simulink model "x3DOF_bener"  (R2024b)
settings: Solver=VariableStepAuto  StartTime=0.0  StopTime=250  FixedStep=au  RelTol=1e-10
undefined symbols (not defined in the file): controller, dr2, dr3, du2, du3, dv2, dv3, gamma, Gpi, guidance, IzMinNrd, m, magnitude, Nr, x_8, x_custom, x_elips, x_L, x_ling, x_s, x_sinus, Xu, Xud, y_8, y_custom, y_elips, y_L, y_ling, y_s, y_sinus, Yv, Yvd
libraries: fuzblock x8, simulink x6, mssSimulink x1
(part 1 of 2)
settings Model: PacingRate=1000  Creator=Baha'uddin  LastModifiedBy=User
settings DebuggingCC: UnderSpecifiedDimensionMsg=error

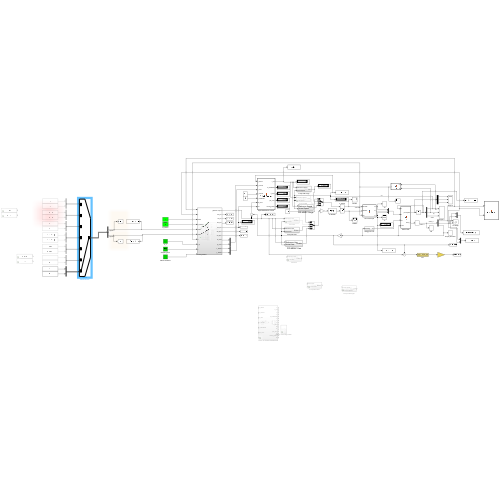
[thumbnail: Simulink's stored preview of the top-level diagram]
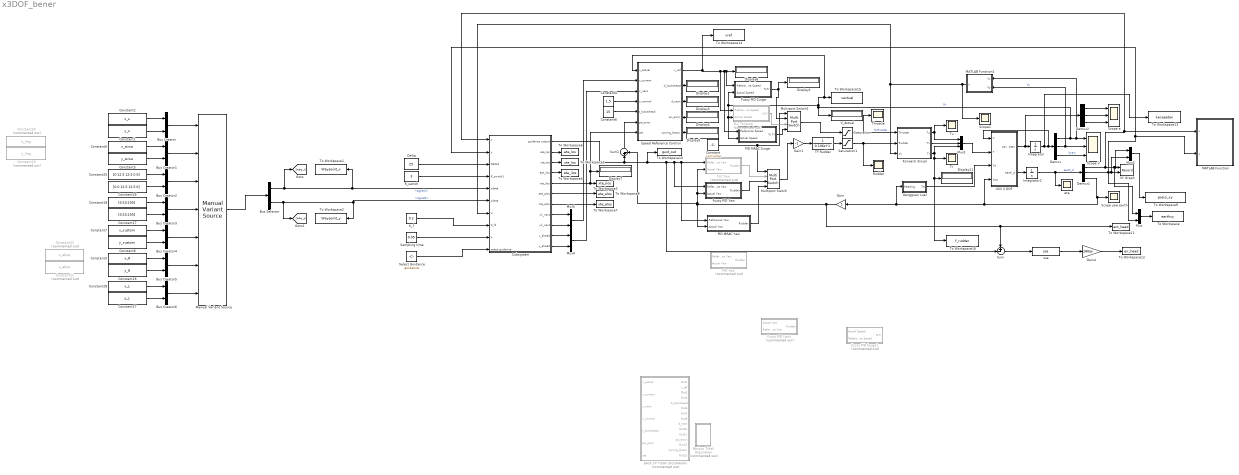
== system x3DOF_bener ==
  BACK UP TIDAK DIGUNAKAN : Subsystem  Commented=on
  Backup Tidak Digunakan : Subsystem  Commented=on
  Bus Creator{,1..6} (7 alike) : BusCreator  Inputs=2
  Bus Selector : BusSelector  OutputSignals=signal1,signal2
  Constant : Constant  Value=controller
  Constant1 : Constant  Value=y_s
  Constant16 : Constant  Value=y_8
  Constant17 : Constant  Value=[0:10:150]
  Constant18 : Constant  Value=[0:10:150]
  Constant2 : Constant  Value=x_s
  Constant21 : Constant  Commented=on  Value=y_elips
  Constant22 : Constant  Commented=on  Value=x_elips
  Constant23 : Constant  Commented=on  Value=y_ling
  Constant24 : Constant  Commented=on  Value=x_ling
  Constant25 : Constant  Value=[0 12.5 12.5 0 0]  VectorParams1D=off
  Constant26 : Constant  Value=[0 0 12.5 12.5 0]
  Constant27 : Constant  Value=y_L
  Constant28 : Constant  Value=x_L
  Constant3 : Constant  Value=x_8
  Constant4 : Constant  Value=1.5
  Constant5 : Constant  Value=y_sinus
  Constant6 : Constant  Value=15
  Constant7 : Constant  Value=x_custom
  Constant8 : Constant  Value=y_custom
  Constant9 : Constant  Value=x_sinus
  Delta : Constant  Value=25
  Demux : Demux  Outputs=3
  Demux1 : Demux  Outputs=3
  Demux2 : Demux  Outputs=3
  Display{1..7,11} (8 alike) : Display
  FLC Throttle : Subsystem  Commented=on
  FLC Yaw : Subsystem  Commented=on
  Fuzzy PID Surge : Subsystem
  Fuzzy PID Surge1 : Subsystem  Commented=on
  Fuzzy PID Yaw : Subsystem
  Fuzzy PID Yaw1 : Subsystem  Commented=on
  Gain : Gain
  Gain1 : Gain  Gain=-1
  Gain4 : Gain  Gain=180/pi
  Gangguan Luar : Subsystem
  Integrator : Integrator  InitialCondition=[0 0 0]
  Integrator2 : Integrator  InitialCondition=[0 0 deg2rad(0)]
  K_f : Constant  Value=0.2
  "Konversi Sinyal " : MATLAB Function  TreatAsAtomicUnit=on
  MATLAB Function : MATLAB Function  TreatAsAtomicUnit=on  SystemSampleTime=0.1
  MATLAB Function1 : MATLAB Function  TreatAsAtomicUnit=on
  Manual Variant Source : simulink/Signal Routing/Manual Variant Source  NumChoices=7  LabelModeActiveChoice=V_7
  Multiport Switch : MultiPortSwitch  SaturateOnIntegerOverflow=off  InputSameDT=off
  Multiport Switch1 : MultiPortSwitch  SaturateOnIntegerOverflow=off  InputSameDT=off
  Mux{,3..5} (4 alike) : Mux  Inputs=2
  Mux1 : Mux  Inputs=3
  PID MRAC Surge : Subsystem
  PID MRAC Yaw : Subsystem
  PID Yaw : Subsystem  Commented=on
  R_switch : Constant  Value=3
  Rudder : Scope
  Sampling time : Constant  Value=0.05
  Saturation : Saturate  UpperLimit=100  LowerLimit=0  ZeroCross=off
  Saturation1 : Saturate  UpperLimit=deg2rad(30)  LowerLimit=deg2rad(-30)
  Scope V : Scope  NumInputPorts=3
  Scope a : Scope  NumInputPorts=3
  Scope yaw earth : Scope
  Scope1 : Scope
  Select Guidance : Constant  Value=guidance
  Speed Reference Control : MATLAB Function  TreatAsAtomicUnit=on
  Subsystem : Subsystem
  Sum : Sum  Inputs=+-|
  Sum1 : Sum  Inputs=|+-
  TF Rudder : TransferFcn  Denominator=[0.106 1]
  Throttle : Scope
  To Workspace : ToWorkspace  VariableName=earthxy  SampleTime=-1
  To Workspace1 : ToWorkspace  VariableName=Waypoint_x  SampleTime=-1
  To Workspace10 : ToWorkspace  VariableName=guid_out  SaveFormat=Timeseries  SampleTime=0.05
      settings: Save2DSignal=2-D array (concatenate along first dimension)
  To Workspace11 : ToWorkspace  VariableName=act_head  SaveFormat=Timeseries  SampleTime=0.05
      settings: Save2DSignal=2-D array (concatenate along first dimension)
  To Workspace12 : ToWorkspace  VariableName=err_head  SaveFormat=Timeseries  SampleTime=0.05
      settings: Save2DSignal=2-D array (concatenate along first dimension)
  To Workspace13 : ToWorkspace  VariableName=kecepatan  SampleTime=1
  To Workspace14 : ToWorkspace  VariableName=vref  SampleTime=0.01
  To Workspace15 : ToWorkspace  VariableName=vactual  SampleTime=0.01
  To Workspace16 : ToWorkspace  VariableName=f_rudder  SampleTime=1
  To Workspace2 : ToWorkspace  VariableName=Waypoint_y  SampleTime=-1
  To Workspace3 : ToWorkspace  VariableName=xte_ilos  SaveFormat=Timeseries  SampleTime=0.05
  To Workspace4 : ToWorkspace  VariableName=ate_ilos  SaveFormat=Timeseries  SampleTime=0.05
  To Workspace5 : ToWorkspace  VariableName=xte_los  SaveFormat=Timeseries  SampleTime=0.05
      settings: Save2DSignal=2-D array (concatenate along first dimension)
  To Workspace6 : ToWorkspace  VariableName=ate_los  SaveFormat=Timeseries  SampleTime=0.05
      settings: Save2DSignal=2-D array (concatenate along first dimension)
  To Workspace7 : ToWorkspace  VariableName=xte_alos  SaveFormat=Timeseries  SampleTime=0.05
      settings: Save2DSignal=2-D array (concatenate along first dimension)
  To Workspace8 : ToWorkspace  VariableName=ate_alos  SaveFormat=Timeseries  SampleTime=0.05
      settings: Save2DSignal=2-D array (concatenate along first dimension)
  To Workspace9 : ToWorkspace  VariableName=posisi_xy  SampleTime=-1
      settings: Save2DSignal=2-D array (concatenate along first dimension)
  Tr : Scope
  Tu : Scope
  USV 3 DOF : MATLAB Function  TreatAsAtomicUnit=on
  V_Actual : Display
  XY Graph : Record  FileSettingsInternal="{\"entries\":[{\"content\":{\"excelSettings\":{\"content\":{},\"type\":\"Streamout.ExcelSettings\"}},\"type\":\"Streamout.FileSettingStorage\",\"uuid\":\"\"}],\"packageUris\":[\"http:\\/\\/schema.mathworks.com\\/mf0\\/streamout_blocks\\/R2020a\"],\"version\":\"1.0\"}"  Layout=[1 1]  SignalsInternal="{\"entries\":[{\"content\":{\"signals\":[{\"content\":{\"blockPath\":[],\"dimensions\":[1],\"domain\":\"\",\"lineColor\":\"#a2142f\",\"lineWidth\":2,\"port\":1,\"sid\":[\"\"],\"signalID\":1,\"signalName\":\"Demux1:1\"},\"type\":\"RecordBlkView.Signal\",\"uuid\":\"\"},{\"content\":{\"blockPath\":[],\"dimensions\":[1],\"domain\":\"\",\"lineColor\":\"#139fff\",\"lineWidth\":2,\"port\":2,\"sid\":[\"\"],\"signalID\":2,\"signalName\":\"Demux1:2\"},\"type\":\"RecordBlkView.Signal\",\"uuid\":\"\"}]},\"type\":\"RecordBlkView.InputSignals\",\"uuid\":\"\"}],\"packageUris\":[\"http:\\/\\/schema.mathworks.com\\/mf0\\/streamout_blocks\\/R2020a\"],\"version\":\"1.0\"}"  VisualizationBindings="{\"xyplotplugin\":{\"info\":[{\"series\":[],\"subplotID\":1}]}}"  CompatibilityTag=XY  st=-1
  eta : Scope
  "ssa " : mssSimulink/Utilities/Math Operations/ssa  SystemSampleTime=-1  VariantActivationTime=update diagram  AllowFlexibleInterface=on  Latency=0  AutoFrameSizeCalculation=off
  wires:
  Demux/3 -> Scope V/3  "Vyaw"
  Gangguan Luar/1(Te) -> USV 3 DOF/3(Te)
  USV 3 DOF/2(earth_d) -> Integrator2/1
  "Konversi Sinyal "/2(Tv) -> Mux1/2
  Mux1/1 -> USV 3 DOF/2(T)
  "Konversi Sinyal "/1(Tu) -> Mux1/1, Tu/1
  Integrator/1 -> To Workspace13/1, USV 3 DOF/1(V), Demux/1
  Demux/2 -> MATLAB Function1/2(Vy), Scope V/2  "Vy"
  Integrator2/1 -> Demux1/1, eta/1  "earth_d"
  "Konversi Sinyal "/3(Tr) -> To Workspace16/1, Display11/1, Tr/1, Mux1/3
  Saturation1/1 -> "Konversi Sinyal "/2(Rudder), Rudder/1
  Saturation/1 -> "Konversi Sinyal "/1(Throttle), Throttle/1  "%Throttle"
  USV 3 DOF/1(percepatan) -> Demux2/1, Integrator/1
  Demux2/1 -> Scope a/1
  Demux2/2 -> Scope a/2
  Demux2/3 -> Scope a/3
  Mux/1 -> To Workspace/1
  Gain/1 -> Sum/1, To Workspace11/1, PID MRAC Yaw/2(Actual Yaw), Sum1/2, FLC Yaw/2(Actual Yaw), Fuzzy PID Yaw/2(Actual Yaw)
  Subsystem/6(ate_alos) -> To Workspace8/1
  Subsystem/3(xte_los) -> To Workspace5/1
  Subsystem/7(xte_alos) -> To Workspace7/1
  Subsystem/4(ate_ilos) -> To Workspace4/1
  Subsystem/5(xte_ilos) -> Speed Reference Control/7(cte), Display7/1, To Workspace3/1
  Subsystem/2(ate_los) -> To Workspace6/1
  R_switch/1 -> Subsystem/4(R_switch1)
  K_f/1 -> Subsystem/8(K_f1)
  Delta/1 -> Subsystem/3(Delta1)
  Select Guidance/1 -> Subsystem/10(select guidance)
  Sampling time/1 -> Subsystem/9(h)
  Bus Selector/1 -> [way_x], To Workspace1/1, Subsystem/5(xdata)  "<signal1>"
  Bus Selector/2 -> [way_y], Subsystem/6(ydata), To Workspace2/1  "<signal2>"
  MATLAB Function1/1(y) -> "Konversi Sinyal "/3(Vx), Subsystem/7(U), Scope1/1
  Mux3/1 -> To Workspace9/1
  "ssa "/1 -> Gain4/1
  Gain4/1 -> To Workspace12/1
  Sum/1 -> "ssa "/1
  TF Rudder/1 -> Saturation1/1
  Demux/1 -> Speed Reference Control/1(v_actual), To Workspace15/1, PID MRAC Surge/2(Actual Speed), FLC Throttle/2(Actual Speed), Fuzzy PID Surge/2(Actual Speed), V_Actual/1, MATLAB Function1/1(Vx), Scope V/1  "Vx"
  Subsystem/10(x_ahead) -> Mux4/1
  Subsystem/11(y_ahead) -> Mux4/2
  Subsystem/8(xk_next) -> Mux5/1
  Subsystem/9(yk_next) -> Mux5/2
  Demux1/2 -> Subsystem/2(y), MATLAB Function/2(y), Mux/2, Mux3/2, XY Graph/2
  Subsystem/1(guidance output) -> To Workspace10/1, Sum/2, PID MRAC Yaw/1(Reference Yaw), FLC Yaw/1(Reference Yaw), Fuzzy PID Yaw/1(Reference Yaw), Sum1/1
  Demux1/3 -> USV 3 DOF/4(Yaw), Gain/1, Gangguan Luar/1(Heading), Scope yaw earth/1
  Demux1/1 -> Subsystem/1(x), MATLAB Function/1(x), Mux/1, Mux3/1, XY Graph/1
  Sum1/1 -> Speed Reference Control/6("psi_error ")
  Speed Reference Control/1(v_ref) -> FLC Throttle/1(Reference Speed), PID MRAC Surge/1(Reference Speed), Display6/1, Fuzzy PID Surge/1(Reference Speed), To Workspace14/1
  Speed Reference Control/2(d_lookahead) -> Display1/1
  Speed Reference Control/5(turning_factor) -> Display5/1
  Speed Reference Control/4(psi_error) -> Display4/1
  Speed Reference Control/3(d_next) -> Display3/1
  Gain1/1 -> TF Rudder/1
  Mux5/1 -> Speed Reference Control/2(x_current)
  Constant6/1 -> Speed Reference Control/5(t_lookahead)
  Constant4/1 -> Speed Reference Control/4(v_normal)
  Mux4/1 -> Speed Reference Control/3(x_next)
  Constant3/1 -> Bus Creator5/1
  Constant16/1 -> Bus Creator5/2
  Bus Creator1/1 -> Manual Variant Source/2
  Bus Creator2/1 -> Manual Variant Source/3
  Constant25/1 -> Bus Creator2/1
  Constant26/1 -> Bus Creator2/2
  Constant18/1 -> Bus Creator3/1
  Constant17/1 -> Bus Creator3/2
  Bus Creator3/1 -> Manual Variant Source/4
  Constant7/1 -> Bus Creator4/1
  Constant8/1 -> Bus Creator4/2
  Bus Creator4/1 -> Manual Variant Source/5
  Bus Creator5/1 -> Manual Variant Source/6
  Manual Variant Source/1 -> Bus Selector/1
  Bus Creator/1 -> Manual Variant Source/1
  Constant28/1 -> Bus Creator6/1
  Constant27/1 -> Bus Creator6/2
  Bus Creator6/1 -> Manual Variant Source/7
  FLC Yaw/1(Rudder) -> Multiport Switch/2
  Fuzzy PID Yaw/1(Rudder) -> Multiport Switch/3
  Constant/1 -> Multiport Switch1/1, Multiport Switch/1
  Multiport Switch/1 -> Gain1/1
  Fuzzy PID Surge/1(%Tr) -> Multiport Switch1/2, Display2/1
  FLC Throttle/1(%Tr) -> Multiport Switch1/3
  Constant2/1 -> Bus Creator/1
  Constant1/1 -> Bus Creator/2
  Constant9/1 -> Bus Creator1/1
  Constant5/1 -> Bus Creator1/2
  PID MRAC Yaw/1(Rudder) -> Multiport Switch/4
  Multiport Switch1/1 -> Saturation/1
  PID MRAC Surge/1(% Tr) -> Multiport Switch1/4

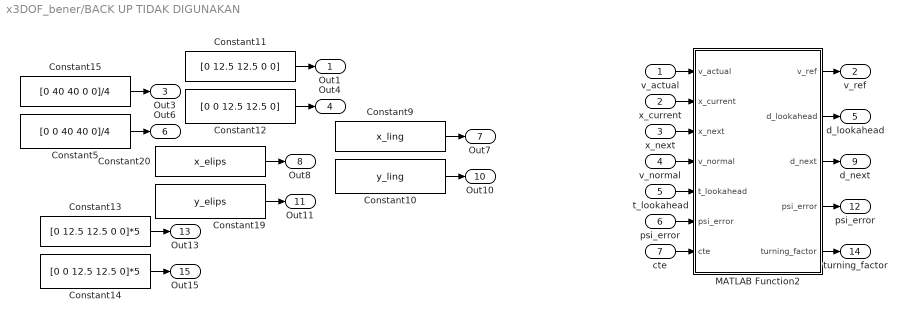
== system x3DOF_bener/BACK UP TIDAK DIGUNAKAN ==
  v_actual : Inport
  x_current : Inport  Port=2
  x_next : Inport  Port=3
  v_normal : Inport  Port=4
  t_lookahead : Inport  Port=5
  "psi_error " : Inport  Port=6
  cte : Inport  Port=7
  Constant10 : Constant  Value=y_ling
  Constant11 : Constant  Value=[0 12.5 12.5 0 0]  VectorParams1D=off
  Constant12 : Constant  Value=[0 0 12.5 12.5 0]
  Constant13 : Constant  Value=[0 12.5 12.5 0 0]*5  VectorParams1D=off
  Constant14 : Constant  Value=[0 0 12.5 12.5 0]*5
  Constant15 : Constant  Value=[0 40 40 0 0]/4  VectorParams1D=off
  Constant19 : Constant  Value=y_elips
  Constant20 : Constant  Value=x_elips
  Constant5 : Constant  Value=[0 0 40 40 0]/4
  Constant9 : Constant  Value=x_ling
  MATLAB Function2 : MATLAB Function  TreatAsAtomicUnit=on
  Out1 : Outport
  v_ref : Outport  Port=2
  Out3 : Outport  Port=3
  Out4 : Outport  Port=4
  d_lookahead : Outport  Port=5
  Out6 : Outport  Port=6
  Out7 : Outport  Port=7
  Out8 : Outport  Port=8
  d_next : Outport  Port=9
  Out10 : Outport  Port=10
  Out11 : Outport  Port=11
  psi_error : Outport  Port=12
  Out13 : Outport  Port=13
  turning_factor : Outport  Port=14
  Out15 : Outport  Port=15
  wires:
  Constant14/1 -> Out15/1
  Constant11/1 -> Out1/1
  Constant9/1 -> Out7/1
  Constant15/1 -> Out3/1
  Constant19/1 -> Out11/1
  Constant5/1 -> Out6/1
  Constant12/1 -> Out4/1
  Constant13/1 -> Out13/1
  Constant20/1 -> Out8/1
  t_lookahead/1 -> MATLAB Function2/5(t_lookahead)
  MATLAB Function2/4(psi_error) -> psi_error/1
  x_current/1 -> MATLAB Function2/2(x_current)
  v_normal/1 -> MATLAB Function2/4(v_normal)
  x_next/1 -> MATLAB Function2/3(x_next)
  "psi_error "/1 -> MATLAB Function2/6("psi_error ")
  cte/1 -> MATLAB Function2/7(cte)
  MATLAB Function2/1(v_ref) -> v_ref/1
  MATLAB Function2/3(d_next) -> d_next/1
  MATLAB Function2/2(d_lookahead) -> d_lookahead/1
  MATLAB Function2/5(turning_factor) -> turning_factor/1
  Constant10/1 -> Out10/1
  v_actual/1 -> MATLAB Function2/1(v_actual)

== system x3DOF_bener/Backup Tidak Digunakan ==
  3 DOF : Subsystem  Commented=on
  From Workspace2 : FromWorkspace  Commented=on  VariableName=THR_ts  SampleTime=0.001
  From Workspace3 : FromWorkspace  Commented=on  VariableName=STER_ts  SampleTime=0.001
  Gangguan Luar1 : Subsystem  Commented=on
  Konversi Sinyal 1 : MATLAB Function  Commented=on  TreatAsAtomicUnit=on
  Mux2 : Mux  Commented=on
  Rudder1 : Scope  Commented=on
  Saturation2 : Saturate  Commented=on  UpperLimit=100  LowerLimit=0
  Saturation3 : Saturate  Commented=on  UpperLimit=35  LowerLimit=-35
  Scope V1 : Scope  Commented=on  NumInputPorts=3
  Scope yaw earth1 : Scope  Commented=on
  TF Rudder1 : TransferFcn  Commented=on  Denominator=[0.106 1]
  ThrCMD1 : Scope  Commented=on
  Tr1 : Scope  Commented=on
  Tu1 : Scope  Commented=on
  VX1 : Scope  Commented=on
  XY Graph1 : Record  Commented=on  FileSettingsInternal="{\"entries\":[{\"content\":{\"excelSettings\":{\"content\":{},\"type\":\"Streamout.ExcelSettings\"}},\"type\":\"Streamout.FileSettingStorage\",\"uuid\":\"\"}],\"packageUris\":[\"http:\\/\\/schema.mathworks.com\\/mf0\\/streamout_blocks\\/R2020a\"],\"version\":\"1.0\"}"  Layout=[1 1]  SignalsInternal="{\"entries\":[{\"content\":{},\"type\":\"RecordBlkView.InputSignals\",\"uuid\":\"\"}],\"packageUris\":[\"http:\\/\\/schema.mathworks.com\\/mf0\\/streamout_blocks\\/R2020a\"],\"version\":\"1.0\"}"  VisualizationBindings="{\"xyplotplugin\":{\"info\":[{\"series\":[],\"subplotID\":1}]}}"  CompatibilityTag=XY  st=-1
  wires:
  3 DOF/1(Out1) -> Scope V1/1, Konversi Sinyal 1/3(Vx), VX1/1  "Vx"
  Mux2/1 -> 3 DOF/1(Input)
  Saturation3/1 -> Konversi Sinyal 1/2(Rudder), Rudder1/1
  Saturation2/1 -> ThrCMD1/1, Konversi Sinyal 1/1(Throttle)
  3 DOF/4(Out4) -> XY Graph1/1
  Konversi Sinyal 1/1(Tu) -> Tu1/1, Mux2/1
  Konversi Sinyal 1/3(Tr) -> Tr1/1, Mux2/3
  3 DOF/5(Out5) -> XY Graph1/2
  Konversi Sinyal 1/2(Tv) -> Mux2/2
  From Workspace3/1 -> Saturation3/1
  Gangguan Luar1/1(Te) -> Mux2/4
  From Workspace2/1 -> Saturation2/1
  3 DOF/3(Out3) -> Scope V1/3  "Vyaw"
  3 DOF/2(Out2) -> Scope V1/2  "Vy"
  3 DOF/6(Out6) -> Gangguan Luar1/1(Heading), Scope yaw earth1/1

== system x3DOF_bener/FLC Throttle ==
  Reference Speed : Inport
  Actual Speed : Inport  Port=2
  Derivative : Derivative
  FLC Thr : fuzblock/Fuzzy Logic  Controller  FIS='FLC_Delta_Gain_Propeller_new.fis'  OutputSampleNumber=101  DataType=double  FuzzifiedInputs=off  RuleFiringStrengths=off  RuleOutputs=off  AggregatedOutputs=off  SimulateUsing=Code generation  OutOfRangeInputValueMessage=warning  NoRuleFiredMessage=warning  EmptyOutputFuzzySetMessage=warning
  FLC Thr1 : fuzblock/Fuzzy Logic  Controller  FIS='FLC_Delta_Gain_Propeller_new_1.fis'  OutputSampleNumber=101  DataType=double  FuzzifiedInputs=off  RuleFiringStrengths=off  RuleOutputs=off  AggregatedOutputs=off  SimulateUsing=Code generation  OutOfRangeInputValueMessage=warning  NoRuleFiredMessage=warning  EmptyOutputFuzzySetMessage=warning
  Manual Variant Sink : simulink/Signal Routing/Manual Variant Sink  NumChoices=2  LabelModeActiveChoice=V_1
  Manual Variant Source : simulink/Signal Routing/Manual Variant Source  NumChoices=2  LabelModeActiveChoice=V_1
  Mux : Mux  Inputs=2
  Scope1 : Scope
  Scope2 : Scope
  Sum : Sum  Inputs=|+-
  %Tr : Outport
  wires:
  Derivative/1 -> Mux/2  "Delta Error"
  Sum/1 -> Scope2/1, Derivative/1, Mux/1  "Error"
  Actual Speed/1 -> Sum/2
  Reference Speed/1 -> Sum/1
  FLC Thr/1 -> Manual Variant Source/2
  Manual Variant Sink/1 -> FLC Thr1/1
  Manual Variant Sink/2 -> FLC Thr/1
  FLC Thr1/1 -> Manual Variant Source/1
  Manual Variant Source/1 -> Scope1/1, %Tr/1
  Mux/1 -> Manual Variant Sink/1

== system x3DOF_bener/FLC Yaw ==
  Reference Yaw : Inport
  Actual Yaw : Inport  Port=2
  Derivative : Derivative
  FLC Yaw : fuzblock/Fuzzy Logic  Controller  FIS='FLC_Delta_Gain_Rudder_new_5MF_tri.fis'  OutputSampleNumber=101  DataType=double  FuzzifiedInputs=off  RuleFiringStrengths=off  RuleOutputs=off  AggregatedOutputs=off  SimulateUsing=Code generation  OutOfRangeInputValueMessage=warning  NoRuleFiredMessage=warning  EmptyOutputFuzzySetMessage=warning
  FLC Yaw 5MF : fuzblock/Fuzzy Logic  Controller  FIS='FLC_Delta_Gain_Rudder_new_5MF_tri_2.fis'  OutputSampleNumber=101  DataType=double  FuzzifiedInputs=off  RuleFiringStrengths=off  RuleOutputs=off  AggregatedOutputs=off  SimulateUsing=Code generation  OutOfRangeInputValueMessage=warning  NoRuleFiredMessage=warning  EmptyOutputFuzzySetMessage=warning
  MATLAB Function1 : MATLAB Function  TreatAsAtomicUnit=on
  Manual Variant Sink : simulink/Signal Routing/Manual Variant Sink  NumChoices=2  LabelModeActiveChoice=V_2
  Manual Variant Source : simulink/Signal Routing/Manual Variant Source  NumChoices=2  LabelModeActiveChoice=V_2
  Mux : Mux  Inputs=2
  Sum : Sum  Inputs=|-+
  Rudder : Outport
  wires:
  Reference Yaw/1 -> MATLAB Function1/1(Reference), Sum/2
  Sum/1 -> MATLAB Function1/2(Error_In)  "Error"
  MATLAB Function1/1(Error) -> Mux/1, Derivative/1
  Actual Yaw/1 -> Sum/1
  Derivative/1 -> Mux/2  "Delta Error"
  Mux/1 -> Manual Variant Sink/1
  Manual Variant Sink/1 -> FLC Yaw 5MF/1
  Manual Variant Sink/2 -> FLC Yaw/1
  Manual Variant Source/1 -> Rudder/1
  FLC Yaw 5MF/1 -> Manual Variant Source/1
  FLC Yaw/1 -> Manual Variant Source/2

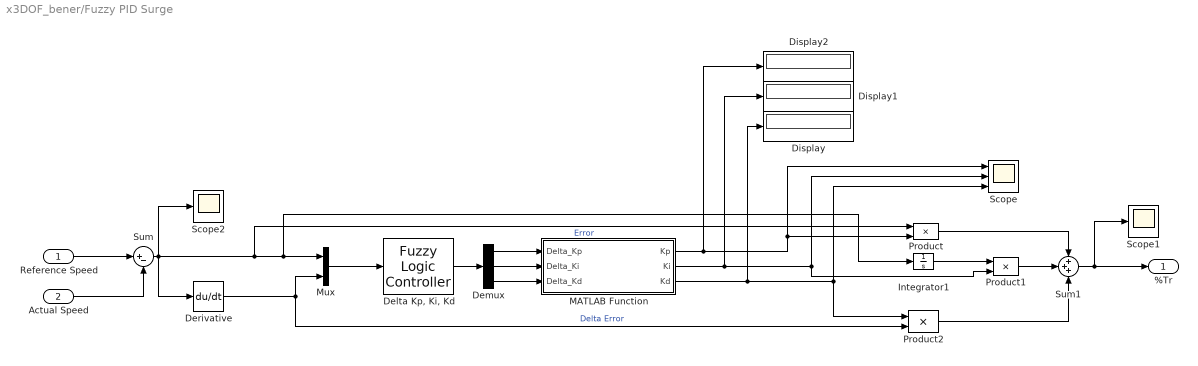
== system x3DOF_bener/Fuzzy PID Surge ==
  Reference Speed : Inport
  Actual Speed : Inport  Port=2
  "Delta Kp, Ki, Kd" : fuzblock/Fuzzy Logic  Controller  FIS='Delta_Gain_Propeller_new.fis'  OutputSampleNumber=101  DataType=double  FuzzifiedInputs=off  RuleFiringStrengths=off  RuleOutputs=off  AggregatedOutputs=off  SimulateUsing=Code generation  OutOfRangeInputValueMessage=warning  NoRuleFiredMessage=warning  EmptyOutputFuzzySetMessage=warning
  Demux : Demux  Outputs=3
  Derivative : Derivative
  Display : Display
  Display1 : Display
  Display2 : Display
  Integrator1 : Integrator
  MATLAB Function : MATLAB Function  TreatAsAtomicUnit=on
  Mux : Mux  Inputs=2
  Product : Product
  Product1 : Product
  Product2 : Product
  Scope : Scope  NumInputPorts=3
  Scope1 : Scope
  Scope2 : Scope
  Sum : Sum  Inputs=|+-
  Sum1 : Sum  Inputs=+++
  %Tr : Outport
  wires:
  Demux/3 -> MATLAB Function/3(Delta_Kd)
  Integrator1/1 -> Product1/1
  Product1/1 -> Sum1/2
  Product2/1 -> Sum1/3
  Product/1 -> Sum1/1
  "Delta Kp, Ki, Kd"/1 -> Demux/1
  Demux/1 -> MATLAB Function/1(Delta_Kp)
  Derivative/1 -> Mux/2, Product2/2  "Delta Error"
  Sum1/1 -> Scope1/1, %Tr/1
  MATLAB Function/3(Kd) -> Display/1, Product2/1, Scope/3
  MATLAB Function/2(Ki) -> Display1/1, Product1/2, Scope/2
  Demux/2 -> MATLAB Function/2(Delta_Ki)
  Mux/1 -> "Delta Kp, Ki, Kd"/1
  MATLAB Function/1(Kp) -> Display2/1, Scope/1, Product/2
  Sum/1 -> Scope2/1, Derivative/1, Product/1, Mux/1, Integrator1/1  "Error"
  Actual Speed/1 -> Sum/2
  Reference Speed/1 -> Sum/1

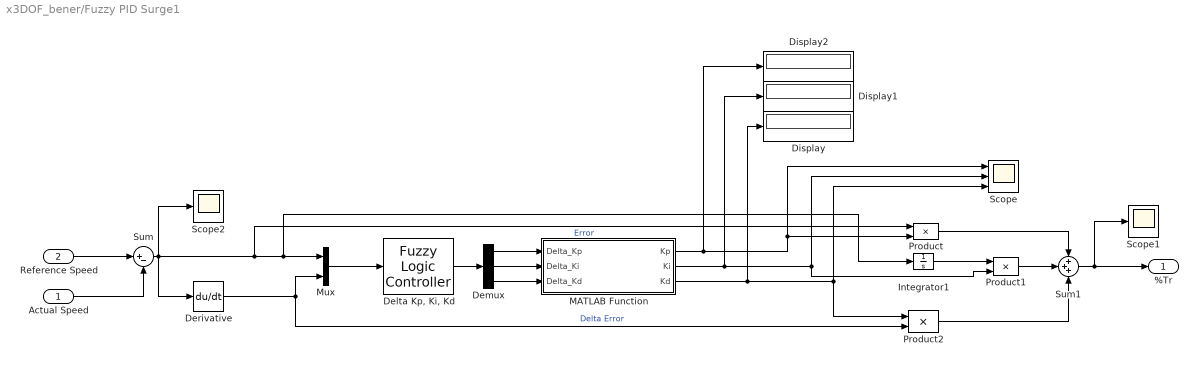
== system x3DOF_bener/Fuzzy PID Surge1 ==
  Actual Speed : Inport
  Reference Speed : Inport  Port=2
  "Delta Kp, Ki, Kd" : fuzblock/Fuzzy Logic  Controller  FIS='Delta_Gain_Propeller_new.fis'  OutputSampleNumber=101  DataType=double  FuzzifiedInputs=off  RuleFiringStrengths=off  RuleOutputs=off  AggregatedOutputs=off  SimulateUsing=Code generation  OutOfRangeInputValueMessage=warning  NoRuleFiredMessage=warning  EmptyOutputFuzzySetMessage=warning
  Demux : Demux  Outputs=3
  Derivative : Derivative
  Display : Display
  Display1 : Display
  Display2 : Display
  Integrator1 : Integrator
  MATLAB Function : MATLAB Function  TreatAsAtomicUnit=on
  Mux : Mux  Inputs=2
  Product : Product
  Product1 : Product
  Product2 : Product
  Scope : Scope  NumInputPorts=3
  Scope1 : Scope
  Scope2 : Scope
  Sum : Sum  Inputs=|+-
  Sum1 : Sum  Inputs=+++
  %Tr : Outport
  wires:
  Demux/3 -> MATLAB Function/3(Delta_Kd)
  Integrator1/1 -> Product1/1
  Product1/1 -> Sum1/2
  Product2/1 -> Sum1/3
  Product/1 -> Sum1/1
  "Delta Kp, Ki, Kd"/1 -> Demux/1
  Demux/1 -> MATLAB Function/1(Delta_Kp)
  Derivative/1 -> Mux/2, Product2/2  "Delta Error"
  Sum1/1 -> Scope1/1, %Tr/1
  MATLAB Function/3(Kd) -> Display/1, Product2/1, Scope/3
  MATLAB Function/2(Ki) -> Display1/1, Product1/2, Scope/2
  Demux/2 -> MATLAB Function/2(Delta_Ki)
  Mux/1 -> "Delta Kp, Ki, Kd"/1
  MATLAB Function/1(Kp) -> Display2/1, Scope/1, Product/2
  Sum/1 -> Scope2/1, Derivative/1, Product/1, Mux/1, Integrator1/1  "Error"
  Actual Speed/1 -> Sum/2
  Reference Speed/1 -> Sum/1

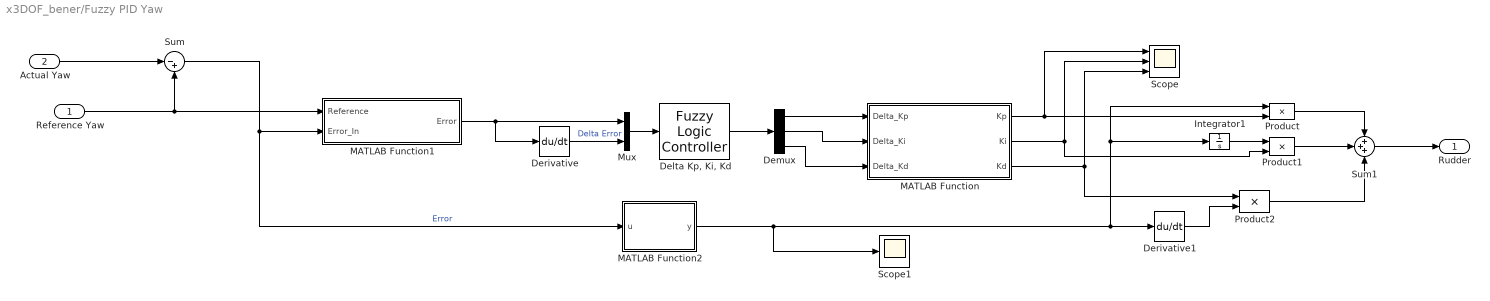
== system x3DOF_bener/Fuzzy PID Yaw ==
  Reference Yaw : Inport
  Actual Yaw : Inport  Port=2
  "Delta Kp, Ki, Kd" : fuzblock/Fuzzy Logic  Controller  FIS='Delta_Gain_Rudder_new.fis'  OutputSampleNumber=101  DataType=double  FuzzifiedInputs=off  RuleFiringStrengths=off  RuleOutputs=off  AggregatedOutputs=off  SimulateUsing=Code generation  OutOfRangeInputValueMessage=warning  NoRuleFiredMessage=warning  EmptyOutputFuzzySetMessage=warning
  Demux : Demux  Outputs=3
  Derivative : Derivative
  Derivative1 : Derivative
  Integrator1 : Integrator
  MATLAB Function : MATLAB Function  TreatAsAtomicUnit=on
  MATLAB Function1 : MATLAB Function  TreatAsAtomicUnit=on
  MATLAB Function2 : MATLAB Function  TreatAsAtomicUnit=on
  Mux : Mux  Inputs=2
  Product : Product
  Product1 : Product
  Product2 : Product
  Scope : Scope  NumInputPorts=3
  Scope1 : Scope
  Sum : Sum  Inputs=|-+
  Sum1 : Sum  Inputs=+++
  Rudder : Outport
  wires:
  MATLAB Function1/1(Error) -> Mux/1, Derivative/1
  Demux/3 -> MATLAB Function/3(Delta_Kd)
  Derivative1/1 -> Product2/2
  Integrator1/1 -> Product1/1
  Derivative/1 -> Mux/2  "Delta Error"
  "Delta Kp, Ki, Kd"/1 -> Demux/1
  Sum1/1 -> Rudder/1
  Demux/2 -> MATLAB Function/2(Delta_Ki)
  Product1/1 -> Sum1/2
  Product/1 -> Sum1/1
  Actual Yaw/1 -> Sum/1
  MATLAB Function/2(Ki) -> Product1/2, Scope/2
  MATLAB Function/1(Kp) -> Product/2, Scope/1
  Demux/1 -> MATLAB Function/1(Delta_Kp)
  Product2/1 -> Sum1/3
  MATLAB Function/3(Kd) -> Product2/1, Scope/3
  Mux/1 -> "Delta Kp, Ki, Kd"/1
  Reference Yaw/1 -> MATLAB Function1/1(Reference), Sum/2
  Sum/1 -> MATLAB Function2/1(u), MATLAB Function1/2(Error_In)  "Error"
  MATLAB Function2/1(y) -> Scope1/1, Product/1, Integrator1/1, Derivative1/1

== system x3DOF_bener/Fuzzy PID Yaw1 ==
  Actual Yaw : Inport
  Reference Yaw : Inport  Port=2
  "Delta Kp, Ki, Kd" : fuzblock/Fuzzy Logic  Controller  FIS='Delta_Gain_Rudder_new.fis'  OutputSampleNumber=101  DataType=double  FuzzifiedInputs=off  RuleFiringStrengths=off  RuleOutputs=off  AggregatedOutputs=off  SimulateUsing=Code generation  OutOfRangeInputValueMessage=warning  NoRuleFiredMessage=warning  EmptyOutputFuzzySetMessage=warning
  Demux : Demux  Outputs=3
  Derivative : Derivative
  Derivative1 : Derivative
  Integrator1 : Integrator
  MATLAB Function : MATLAB Function  TreatAsAtomicUnit=on
  MATLAB Function1 : MATLAB Function  TreatAsAtomicUnit=on
  MATLAB Function2 : MATLAB Function  TreatAsAtomicUnit=on
  Mux : Mux  Inputs=2
  Product : Product
  Product1 : Product
  Product2 : Product
  Scope : Scope  NumInputPorts=3
  Scope1 : Scope
  Sum : Sum  Inputs=|-+
  Sum1 : Sum  Inputs=+++
  Rudder : Outport
  wires:
  MATLAB Function1/1(Error) -> Mux/1, Derivative/1
  Demux/3 -> MATLAB Function/3(Delta_Kd)
  Derivative1/1 -> Product2/2
  Integrator1/1 -> Product1/1
  Derivative/1 -> Mux/2  "Delta Error"
  "Delta Kp, Ki, Kd"/1 -> Demux/1
  Sum1/1 -> Rudder/1
  Demux/2 -> MATLAB Function/2(Delta_Ki)
  Product1/1 -> Sum1/2
  Product/1 -> Sum1/1
  Actual Yaw/1 -> Sum/1
  MATLAB Function/2(Ki) -> Product1/2, Scope/2
  MATLAB Function/1(Kp) -> Product/2, Scope/1
  Demux/1 -> MATLAB Function/1(Delta_Kp)
  Product2/1 -> Sum1/3
  MATLAB Function/3(Kd) -> Product2/1, Scope/3
  Mux/1 -> "Delta Kp, Ki, Kd"/1
  Reference Yaw/1 -> MATLAB Function1/1(Reference), Sum/2
  Sum/1 -> MATLAB Function2/1(u), MATLAB Function1/2(Error_In)  "Error"
  MATLAB Function2/1(y) -> Scope1/1, Product/1, Integrator1/1, Derivative1/1

== system x3DOF_bener/Gangguan Luar ==
  Heading : Inport
  Cbeta : Constant  Commented=on  Value=0
  Current Disturbance : Subsystem  Commented=on
  Gain : Gain  Gain=0
  Mux5 : Mux  Commented=on  Inputs=3
  Mux6 : Mux  Inputs=3
  Mux7 : Mux  Commented=on  Inputs=3
  Sum1 : Sum  Commented=on  Inputs=|++
  Vc : Constant  Commented=on  Value=0.1
  Vw : Constant  Value=0.1
  WaA : Constant  Commented=on  Value=0.15
  "Wabeta " : Constant  Commented=on  Value=0
  Wave Disturbance : Subsystem  Commented=on
  Wbeta : Constant  Value=0
  Wind Disturbance : Subsystem
  Te : Outport
  wires:
  Wbeta/1 -> Wind Disturbance/2(Beta)
  Vc/1 -> Current Disturbance/1(Vc)
  Cbeta/1 -> Current Disturbance/2(Beta)
  Current Disturbance/1(TeU) -> Mux7/1
  Current Disturbance/2(TeV) -> Mux7/2
  Wind Disturbance/2(TeV) -> Mux6/2
  Wind Disturbance/1(TeU) -> Mux6/1
  Wind Disturbance/3(TeR) -> Mux6/3
  Current Disturbance/3(TeR) -> Mux7/3
  Mux6/1 -> Gain/1
  Wave Disturbance/2(TeV) -> Mux5/2
  Wave Disturbance/1(TeU) -> Mux5/1
  Wave Disturbance/3("TeR ") -> Mux5/3
  "Wabeta "/1 -> Wave Disturbance/2(Beta)
  WaA/1 -> Wave Disturbance/1(WaA)
  Vw/1 -> Wind Disturbance/1(Vw)
  Heading/1 -> Wind Disturbance/3(Yaw), Wave Disturbance/3(Yaw), Current Disturbance/3(Yaw)
  Gain/1 -> Te/1
  Mux5/1 -> Sum1/2
  Mux7/1 -> Sum1/1

== system x3DOF_bener/PID MRAC Surge ==
  Reference Speed : Inport
  Actual Speed : Inport  Port=2
  Clock : Clock
  Gain_D1 : Constant  Value=1.5
  Gain_I1 : Constant
  Gain_P : Constant  Value=20
  Mux : Mux  Inputs=7
  PID_MRAC_Diskrit_Translasi : MATLABFcn  MATLABFcn=PID_MRAC_Diskrit_TranslasiTEORI  OutputDimensions=1  OutputSignalType=real  Output1D=off  SampleTime=0.01
  Ts : Constant  Value=0.01
  % Tr : Outport  VectorParamsAs1DForOutWhenUnconnected=off
  wires:
  Mux/1 -> PID_MRAC_Diskrit_Translasi/1
  PID_MRAC_Diskrit_Translasi/1 -> % Tr/1
  Reference Speed/1 -> Mux/1
  Actual Speed/1 -> Mux/2
  Clock/1 -> Mux/7
  Ts/1 -> Mux/6
  Gain_P/1 -> Mux/3
  Gain_I1/1 -> Mux/4
  Gain_D1/1 -> Mux/5

== system x3DOF_bener/PID MRAC Yaw ==
  Reference Yaw : Inport
  Actual Yaw : Inport  Port=2
  Clock : Clock
  Gain_D1 : Constant  Value=3
  Gain_D3 : Constant  Value=400
  Gain_I1 : Constant
  Gain_P1 : Constant  Value=20
  Gain_P3 : Constant  Value=150
  Gain_Pfix : Constant  Value=100
  Mux : Mux  Inputs=7
  PID_MRAC_Diskrit_Kemudi : MATLABFcn  MATLABFcn=PID_MRAC_Diskrit_KemudiTEORI  OutputDimensions=1  OutputSignalType=real  Output1D=off  SampleTime=0.01
  Ts : Constant  Value=0.01
  Rudder : Outport  VectorParamsAs1DForOutWhenUnconnected=off
  wires:
  Mux/1 -> PID_MRAC_Diskrit_Kemudi/1
  PID_MRAC_Diskrit_Kemudi/1 -> Rudder/1
  Reference Yaw/1 -> Mux/1
  Actual Yaw/1 -> Mux/2
  Ts/1 -> Mux/6
  Clock/1 -> Mux/7
  Gain_P1/1 -> Mux/3
  Gain_I1/1 -> Mux/4
  Gain_D1/1 -> Mux/5

== system x3DOF_bener/PID Yaw ==
  Reference Yaw : Inport
  Actual Yaw : Inport  Port=2
  Derivative1 : Derivative
  Gain : Gain  Gain=5
  Gain1 : Gain  Gain=0
  Gain2 : Gain  Gain=1.2
  Integrator : Integrator
  MATLAB Function2 : MATLAB Function  TreatAsAtomicUnit=on
  Manual Variant Sink : simulink/Signal Routing/Manual Variant Sink  NumChoices=2  LabelModeActiveChoice=V_1
  Scope : Scope
  Scope1 : Scope
  Sum : Sum  Inputs=|-+
  Sum1 : Sum  Inputs=+++
  To File6 : ToFile  Filename=D:\ITS\S2\Semester 4\Paper Bu Lita\Data\3. Pengujian Sinus\Error_Yaw_PID.mat  MatrixName=eYaw_PID  SampleTime=0.01
  Rudder : Outport
  wires:
  Sum1/1 -> Scope1/1, Rudder/1
  Gain1/1 -> Sum1/2
  Gain/1 -> Sum1/1
  Actual Yaw/1 -> Sum/1
  Reference Yaw/1 -> Sum/2
  Integrator/1 -> Gain1/1
  Derivative1/1 -> Gain2/1
  Gain2/1 -> Sum1/3
  Sum/1 -> Manual Variant Sink/1, MATLAB Function2/1(u)  "Error"
  MATLAB Function2/1(y) -> Gain/1, Scope/1, Derivative1/1, Integrator/1
  Manual Variant Sink/2 -> To File6/1

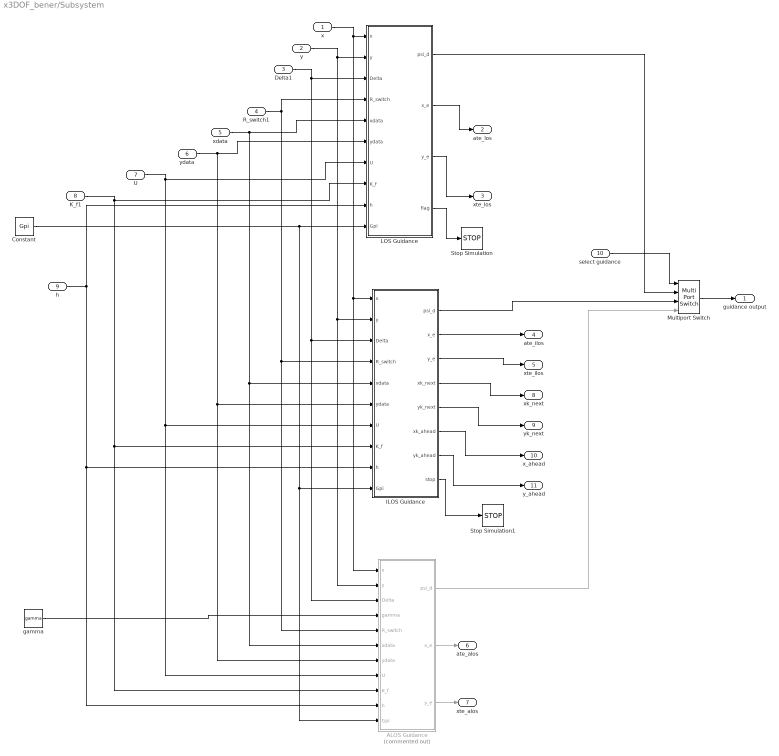
== system x3DOF_bener/Subsystem ==
  x : Inport
  y : Inport  Port=2
  Delta1 : Inport  Port=3
  R_switch1 : Inport  Port=4
  xdata : Inport  Port=5
  ydata : Inport  Port=6
  U : Inport  Port=7
  K_f1 : Inport  Port=8
  h : Inport  Port=9
  select guidance : Inport  Port=10
  ALOS Guidance : MATLAB Function  Commented=on  TreatAsAtomicUnit=on
  Constant : Constant  Value=Gpi
  ILOS Guidance : MATLAB Function  TreatAsAtomicUnit=on
  LOS Guidance : MATLAB Function  TreatAsAtomicUnit=on
  Multiport Switch : MultiPortSwitch  SaturateOnIntegerOverflow=off  InputSameDT=off
  Stop Simulation : Stop
  Stop Simulation1 : Stop
  gamma : Constant  Value=gamma
  guidance output : Outport
  ate_los : Outport  Port=2
  xte_los : Outport  Port=3
  ate_ilos : Outport  Port=4
  xte_ilos : Outport  Port=5
  ate_alos : Outport  Port=6
  xte_alos : Outport  Port=7
  xk_next : Outport  Port=8
  yk_next : Outport  Port=9
  x_ahead : Outport  Port=10
  y_ahead : Outport  Port=11
  wires:
  xdata/1 -> ALOS Guidance/6(xdata), ILOS Guidance/5(xdata), LOS Guidance/5(xdata)
  gamma/1 -> ALOS Guidance/4(gamma)
  Delta1/1 -> ILOS Guidance/3(Delta), ALOS Guidance/3(Delta), LOS Guidance/3(Delta)
  h/1 -> ALOS Guidance/10(h), ILOS Guidance/9(h), LOS Guidance/9(h)
  x/1 -> ALOS Guidance/1(x), ILOS Guidance/1(x), LOS Guidance/1(x)
  K_f1/1 -> ALOS Guidance/9(K_f), ILOS Guidance/8(K_f), LOS Guidance/8(K_f)
  U/1 -> ALOS Guidance/8(U), ILOS Guidance/7(U), LOS Guidance/7(U)
  ydata/1 -> ALOS Guidance/7(ydata), ILOS Guidance/6(ydata), LOS Guidance/6(ydata)
  y/1 -> ILOS Guidance/2(y), ALOS Guidance/2(y), LOS Guidance/2(y)
  R_switch1/1 -> ALOS Guidance/5(R_switch), ILOS Guidance/4(R_switch), LOS Guidance/4(R_switch)
  ALOS Guidance/1(psi_d) -> Multiport Switch/4
  LOS Guidance/1(psi_d) -> Multiport Switch/2
  ILOS Guidance/1(psi_d) -> Multiport Switch/3
  select guidance/1 -> Multiport Switch/1
  Multiport Switch/1 -> guidance output/1
  ILOS Guidance/3(y_e) -> xte_ilos/1
  ILOS Guidance/2(x_e) -> ate_ilos/1
  LOS Guidance/2(x_e) -> ate_los/1
  LOS Guidance/3(y_e) -> xte_los/1
  ALOS Guidance/2(x_e) -> ate_alos/1
  ALOS Guidance/3(y_e) -> xte_alos/1
  LOS Guidance/4(flag) -> Stop Simulation/1
  Constant/1 -> ALOS Guidance/11(Gpi), ILOS Guidance/10(Gpi), LOS Guidance/10(Gpi)
  ILOS Guidance/4(xk_next) -> xk_next/1
  ILOS Guidance/5(yk_next) -> yk_next/1
  ILOS Guidance/7(yk_ahead) -> y_ahead/1
  ILOS Guidance/6(xk_ahead) -> x_ahead/1
  ILOS Guidance/8(stop) -> Stop Simulation1/1

== system x3DOF_bener/Backup Tidak Digunakan/3 DOF ==
  Input : Inport
  Demux : Demux  Outputs=3
  Integrator{,1..3} (4 alike) : Integrator
  MATLAB Function : MATLAB Function  TreatAsAtomicUnit=on
  Mux : Mux  Inputs=3
  Sumbu X : Fcn  Expr=1/(m-Xud)*((m-Yvd)*u(2)*u(3) - Xu*u(1) - du2*abs(u(1))*u(1) - du3*(abs(u(1))^2)*u(1) + u(4))
  Sumbu Y : Fcn  Expr=1/(m-Yvd)*(-(m-Xud)*u(1)*u(3) - Yv*u(2) - dv2*abs(u(2))*u(2) - dv3*(abs(u(2))^2)*u(2))
  Sumbu Yaw : Fcn  Expr=1/(IzMinNrd)*(-(m-Yvd)*u(2)*u(1) + (m-Xud)*u(1)*u(2) - Nr*u(3) - dr2*abs(u(3))*u(3) - dr3*(abs(u(3))^2)*u(3) + u(5))
  Out1 : Outport
  Out2 : Outport  Port=2
  Out3 : Outport  Port=3
  Out4 : Outport  Port=4
  Out5 : Outport  Port=5
  Out6 : Outport  Port=6
  wires:
  Sumbu Yaw/1 -> Integrator2/1
  Sumbu X/1 -> Integrator/1
  Input/1 -> Sumbu Yaw/1, Sumbu Y/1, Sumbu X/1
  Sumbu Y/1 -> Integrator1/1
  Integrator/1 -> Mux/1, Out1/1
  Integrator1/1 -> Mux/2, Out2/1
  Integrator2/1 -> Mux/3, Out3/1
  MATLAB Function/1(eta_d) -> Integrator3/1
  Integrator3/1 -> Demux/1
  Demux/3 -> MATLAB Function/2(Yaw), Out6/1
  Demux/2 -> Out5/1
  Demux/1 -> Out4/1
  Mux/1 -> MATLAB Function/1(V)

== system x3DOF_bener/Backup Tidak Digunakan/Gangguan Luar1 ==
  Heading : Inport
  Cbeta : Constant  Commented=on  Value=0
  Current Disturbance : Subsystem  Commented=on
  Gain : Gain  Gain=0
  Mux5 : Mux  Commented=on  Inputs=3
  Mux6 : Mux  Inputs=3
  Mux7 : Mux  Commented=on  Inputs=3
  Sum1 : Sum  Commented=on  Inputs=|++
  Vc : Constant  Commented=on  Value=0.1
  Vw : Constant  Value=0.1
  WaA : Constant  Commented=on  Value=0.15
  "Wabeta " : Constant  Commented=on  Value=0
  Wave Disturbance : Subsystem  Commented=on
  Wbeta : Constant  Value=0
  Wind Disturbance : Subsystem
  Te : Outport
  wires:
  Wbeta/1 -> Wind Disturbance/2(Beta)
  Vc/1 -> Current Disturbance/1(Vc)
  Cbeta/1 -> Current Disturbance/2(Beta)
  Current Disturbance/1(TeU) -> Mux7/1
  Current Disturbance/2(TeV) -> Mux7/2
  Wind Disturbance/2(TeV) -> Mux6/2
  Wind Disturbance/1(TeU) -> Mux6/1
  Wind Disturbance/3(TeR) -> Mux6/3
  Current Disturbance/3(TeR) -> Mux7/3
  Mux6/1 -> Gain/1
  Wave Disturbance/2(TeV) -> Mux5/2
  Wave Disturbance/1(TeU) -> Mux5/1
  Wave Disturbance/3("TeR ") -> Mux5/3
  "Wabeta "/1 -> Wave Disturbance/2(Beta)
  WaA/1 -> Wave Disturbance/1(WaA)
  Vw/1 -> Wind Disturbance/1(Vw)
  Heading/1 -> Wind Disturbance/3(Yaw), Wave Disturbance/3(Yaw), Current Disturbance/3(Yaw)
  Gain/1 -> Te/1
  Mux5/1 -> Sum1/2
  Mux7/1 -> Sum1/1

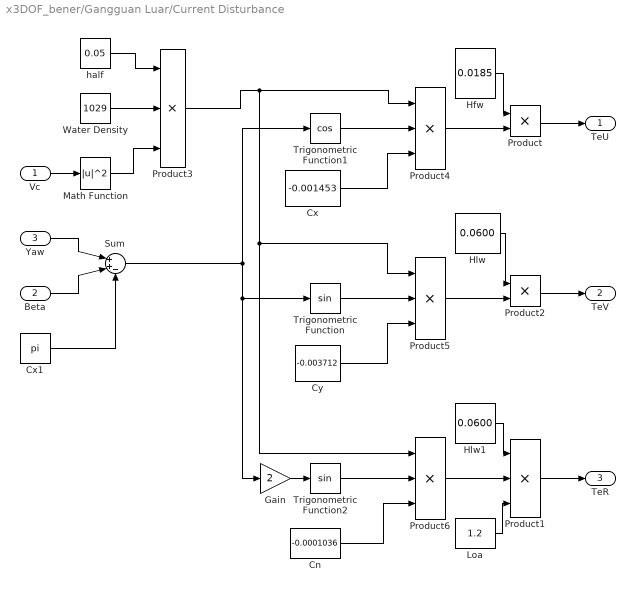
== system x3DOF_bener/Gangguan Luar/Current Disturbance ==
  Vc : Inport
  Beta : Inport  Port=2
  Yaw : Inport  Port=3
  Cn : Constant  Value=-0.0001036
  Cx : Constant  Value=-0.001453
  Cx1 : Constant  Value=pi
  Cy : Constant  Value=-0.003712
  Gain : Gain  Gain=2
  Hfw : Constant  Value=0.0185
  Hlw : Constant  Value=0.0600
  Hlw1 : Constant  Value=0.0600
  Loa : Constant  Value=1.2
  Math Function : Math  Operator=magnitude^2  SignedPower=on
  Product : Product
  Product{1,3..6} (5 alike) : Product  Inputs=3
  Product2 : Product
  Sum : Sum  Inputs=|++-
  Trigonometric Function : Trigonometry
  Trigonometric Function1 : Trigonometry  Operator=cos
  Trigonometric Function2 : Trigonometry
  Water Density : Constant  Value=1029
  half : Constant  Value=0.05
  TeU : Outport
  TeV : Outport  Port=2
  TeR : Outport  Port=3
  wires:
  Vc/1 -> Math Function/1
  Product/1 -> TeU/1
  Hfw/1 -> Product/1
  Product2/1 -> TeV/1
  Hlw/1 -> Product2/1
  Product1/1 -> TeR/1
  Hlw1/1 -> Product1/1
  Loa/1 -> Product1/3
  Yaw/1 -> Sum/1
  Beta/1 -> Sum/2
  Cx1/1 -> Sum/3
  Water Density/1 -> Product3/2
  Math Function/1 -> Product3/3
  half/1 -> Product3/1
  Product4/1 -> Product/2
  Trigonometric Function1/1 -> Product4/2
  Cx/1 -> Product4/3
  Sum/1 -> Trigonometric Function1/1, Gain/1, Trigonometric Function/1
  Product3/1 -> Product6/1, Product5/1, Product4/1
  Product5/1 -> Product2/2
  Trigonometric Function/1 -> Product5/2
  Cy/1 -> Product5/3
  Product6/1 -> Product1/2
  Trigonometric Function2/1 -> Product6/2
  Cn/1 -> Product6/3
  Gain/1 -> Trigonometric Function2/1

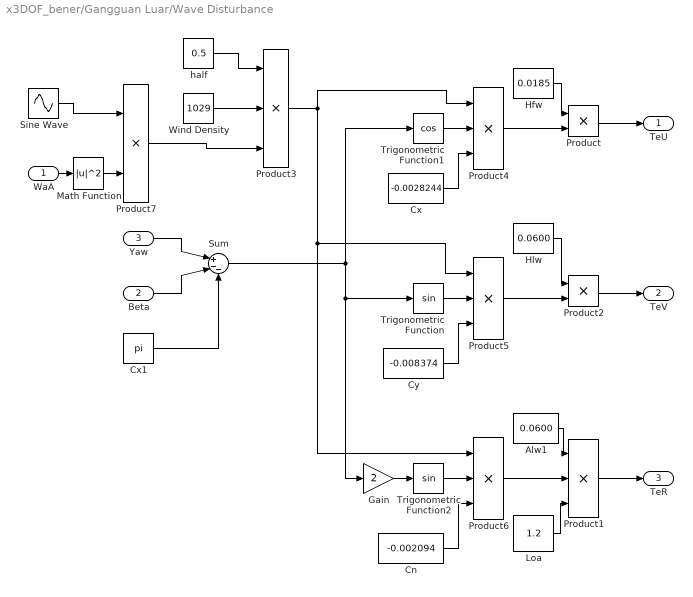
== system x3DOF_bener/Gangguan Luar/Wave Disturbance ==
  WaA : Inport
  Beta : Inport  Port=2
  Yaw : Inport  Port=3
  Alw1 : Constant  Value=0.0600
  Cn : Constant  Value=-0.002094
  Cx : Constant  Value=-0.0028244
  Cx1 : Constant  Value=pi
  Cy : Constant  Value=-0.008374
  Gain : Gain  Gain=2
  Hfw : Constant  Value=0.0185
  Hlw : Constant  Value=0.0600
  Loa : Constant  Value=1.2
  Math Function : Math  Operator=magnitude^2  SignedPower=on
  Product : Product
  Product{1,3..6} (5 alike) : Product  Inputs=3
  Product2 : Product
  Product7 : Product
  Sine Wave : Sin  Amplitude=0.1  Frequency=0.08  SampleTime=0
  Sum : Sum  Inputs=|+--
  Trigonometric Function : Trigonometry
  Trigonometric Function1 : Trigonometry  Operator=cos
  Trigonometric Function2 : Trigonometry
  Wind Density : Constant  Value=1029
  half : Constant  Value=0.5
  TeU : Outport
  TeV : Outport  Port=2
  "TeR " : Outport  Port=3
  wires:
  Product/1 -> TeU/1
  Hfw/1 -> Product/1
  Product2/1 -> TeV/1
  Hlw/1 -> Product2/1
  Product1/1 -> "TeR "/1
  Alw1/1 -> Product1/1
  Loa/1 -> Product1/3
  Yaw/1 -> Sum/1
  Beta/1 -> Sum/2
  Cx1/1 -> Sum/3
  Wind Density/1 -> Product3/2
  half/1 -> Product3/1
  Product4/1 -> Product/2
  Trigonometric Function1/1 -> Product4/2
  Cx/1 -> Product4/3
  Sum/1 -> Trigonometric Function1/1, Gain/1, Trigonometric Function/1
  Product3/1 -> Product4/1, Product6/1, Product5/1
  Product5/1 -> Product2/2
  Trigonometric Function/1 -> Product5/2
  Cy/1 -> Product5/3
  Product6/1 -> Product1/2
  Trigonometric Function2/1 -> Product6/2
  Cn/1 -> Product6/3
  Gain/1 -> Trigonometric Function2/1
  Sine Wave/1 -> Product7/1
  WaA/1 -> Math Function/1
  Math Function/1 -> Product7/2
  Product7/1 -> Product3/3

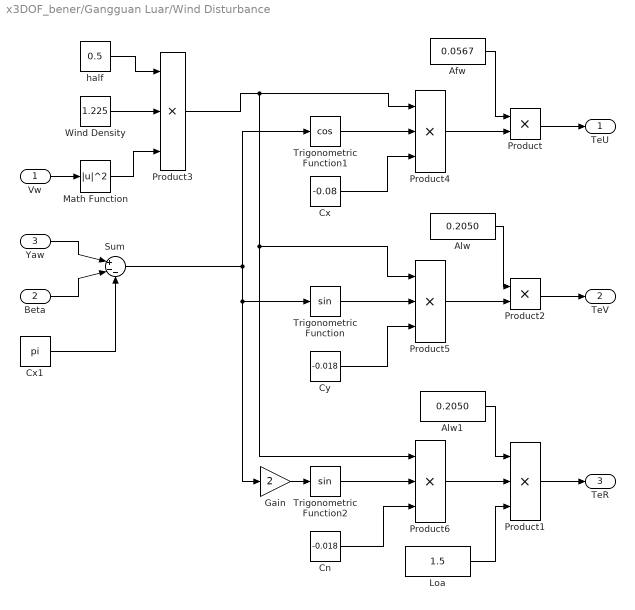
== system x3DOF_bener/Gangguan Luar/Wind Disturbance ==
  Vw : Inport
  Beta : Inport  Port=2
  Yaw : Inport  Port=3
  Afw : Constant  Value=0.0567
  Alw : Constant  Value=0.2050
  Alw1 : Constant  Value=0.2050
  Cn : Constant  Value=-0.018
  Cx : Constant  Value=-0.08
  Cx1 : Constant  Value=pi
  Cy : Constant  Value=-0.018
  Gain : Gain  Gain=2
  Loa : Constant  Value=1.5
  Math Function : Math  Operator=magnitude^2  SignedPower=on
  Product : Product
  Product{1,3..6} (5 alike) : Product  Inputs=3
  Product2 : Product
  Sum : Sum  Inputs=|+--
  Trigonometric Function : Trigonometry
  Trigonometric Function1 : Trigonometry  Operator=cos
  Trigonometric Function2 : Trigonometry
  Wind Density : Constant  Value=1.225
  half : Constant  Value=0.5
  TeU : Outport
  TeV : Outport  Port=2
  TeR : Outport  Port=3
  wires:
  Vw/1 -> Math Function/1
  Product/1 -> TeU/1
  Afw/1 -> Product/1
  Product2/1 -> TeV/1
  Alw/1 -> Product2/1
  Product1/1 -> TeR/1
  Alw1/1 -> Product1/1
  Loa/1 -> Product1/3
  Yaw/1 -> Sum/1
  Beta/1 -> Sum/2
  Cx1/1 -> Sum/3
  Wind Density/1 -> Product3/2
  Math Function/1 -> Product3/3
  half/1 -> Product3/1
  Product4/1 -> Product/2
  Trigonometric Function1/1 -> Product4/2
  Cx/1 -> Product4/3
  Sum/1 -> Trigonometric Function1/1, Gain/1, Trigonometric Function/1
  Product3/1 -> Product6/1, Product5/1, Product4/1
  Product5/1 -> Product2/2
  Trigonometric Function/1 -> Product5/2
  Cy/1 -> Product5/3
  Product6/1 -> Product1/2
  Trigonometric Function2/1 -> Product6/2
  Cn/1 -> Product6/3
  Gain/1 -> Trigonometric Function2/1

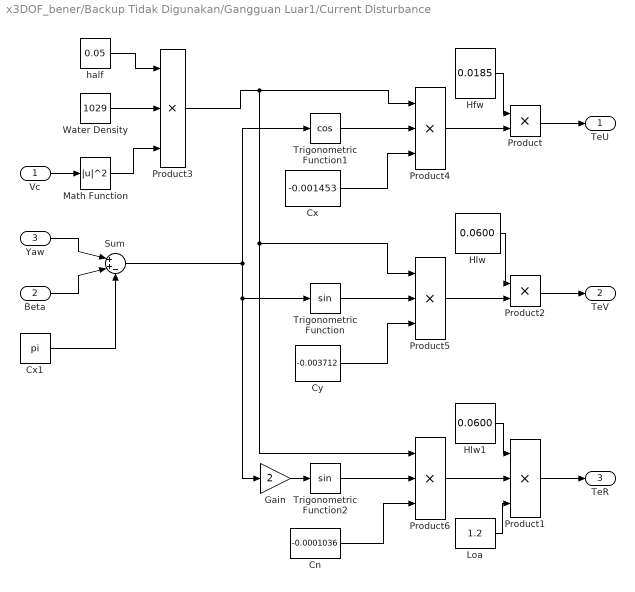
== system x3DOF_bener/Backup Tidak Digunakan/Gangguan Luar1/Current Disturbance ==
  Vc : Inport
  Beta : Inport  Port=2
  Yaw : Inport  Port=3
  Cn : Constant  Value=-0.0001036
  Cx : Constant  Value=-0.001453
  Cx1 : Constant  Value=pi
  Cy : Constant  Value=-0.003712
  Gain : Gain  Gain=2
  Hfw : Constant  Value=0.0185
  Hlw : Constant  Value=0.0600
  Hlw1 : Constant  Value=0.0600
  Loa : Constant  Value=1.2
  Math Function : Math  Operator=magnitude^2  SignedPower=on
  Product : Product
  Product{1,3..6} (5 alike) : Product  Inputs=3
  Product2 : Product
  Sum : Sum  Inputs=|++-
  Trigonometric Function : Trigonometry
  Trigonometric Function1 : Trigonometry  Operator=cos
  Trigonometric Function2 : Trigonometry
  Water Density : Constant  Value=1029
  half : Constant  Value=0.05
  TeU : Outport
  TeV : Outport  Port=2
  TeR : Outport  Port=3
  wires:
  Vc/1 -> Math Function/1
  Product/1 -> TeU/1
  Hfw/1 -> Product/1
  Product2/1 -> TeV/1
  Hlw/1 -> Product2/1
  Product1/1 -> TeR/1
  Hlw1/1 -> Product1/1
  Loa/1 -> Product1/3
  Yaw/1 -> Sum/1
  Beta/1 -> Sum/2
  Cx1/1 -> Sum/3
  Water Density/1 -> Product3/2
  Math Function/1 -> Product3/3
  half/1 -> Product3/1
  Product4/1 -> Product/2
  Trigonometric Function1/1 -> Product4/2
  Cx/1 -> Product4/3
  Sum/1 -> Trigonometric Function1/1, Gain/1, Trigonometric Function/1
  Product3/1 -> Product6/1, Product5/1, Product4/1
  Product5/1 -> Product2/2
  Trigonometric Function/1 -> Product5/2
  Cy/1 -> Product5/3
  Product6/1 -> Product1/2
  Trigonometric Function2/1 -> Product6/2
  Cn/1 -> Product6/3
  Gain/1 -> Trigonometric Function2/1

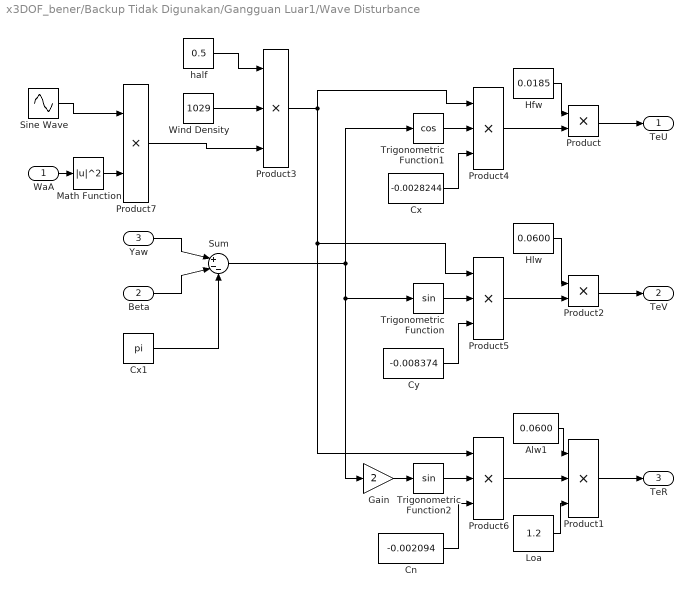
== system x3DOF_bener/Backup Tidak Digunakan/Gangguan Luar1/Wave Disturbance ==
  WaA : Inport
  Beta : Inport  Port=2
  Yaw : Inport  Port=3
  Alw1 : Constant  Value=0.0600
  Cn : Constant  Value=-0.002094
  Cx : Constant  Value=-0.0028244
  Cx1 : Constant  Value=pi
  Cy : Constant  Value=-0.008374
  Gain : Gain  Gain=2
  Hfw : Constant  Value=0.0185
  Hlw : Constant  Value=0.0600
  Loa : Constant  Value=1.2
  Math Function : Math  Operator=magnitude^2  SignedPower=on
  Product : Product
  Product{1,3..6} (5 alike) : Product  Inputs=3
  Product2 : Product
  Product7 : Product
  Sine Wave : Sin  Amplitude=0.1  Frequency=0.08  SampleTime=0
  Sum : Sum  Inputs=|+--
  Trigonometric Function : Trigonometry
  Trigonometric Function1 : Trigonometry  Operator=cos
  Trigonometric Function2 : Trigonometry
  Wind Density : Constant  Value=1029
  half : Constant  Value=0.5
  TeU : Outport
  TeV : Outport  Port=2
  "TeR " : Outport  Port=3
  wires:
  Product/1 -> TeU/1
  Hfw/1 -> Product/1
  Product2/1 -> TeV/1
  Hlw/1 -> Product2/1
  Product1/1 -> "TeR "/1
  Alw1/1 -> Product1/1
  Loa/1 -> Product1/3
  Yaw/1 -> Sum/1
  Beta/1 -> Sum/2
  Cx1/1 -> Sum/3
  Wind Density/1 -> Product3/2
  half/1 -> Product3/1
  Product4/1 -> Product/2
  Trigonometric Function1/1 -> Product4/2
  Cx/1 -> Product4/3
  Sum/1 -> Trigonometric Function1/1, Gain/1, Trigonometric Function/1
  Product3/1 -> Product4/1, Product6/1, Product5/1
  Product5/1 -> Product2/2
  Trigonometric Function/1 -> Product5/2
  Cy/1 -> Product5/3
  Product6/1 -> Product1/2
  Trigonometric Function2/1 -> Product6/2
  Cn/1 -> Product6/3
  Gain/1 -> Trigonometric Function2/1
  Sine Wave/1 -> Product7/1
  WaA/1 -> Math Function/1
  Math Function/1 -> Product7/2
  Product7/1 -> Product3/3

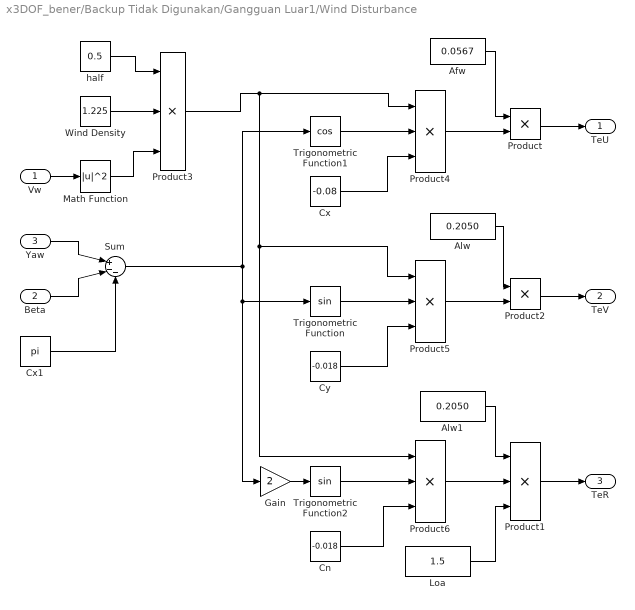
== system x3DOF_bener/Backup Tidak Digunakan/Gangguan Luar1/Wind Disturbance ==
  Vw : Inport
  Beta : Inport  Port=2
  Yaw : Inport  Port=3
  Afw : Constant  Value=0.0567
  Alw : Constant  Value=0.2050
  Alw1 : Constant  Value=0.2050
  Cn : Constant  Value=-0.018
  Cx : Constant  Value=-0.08
  Cx1 : Constant  Value=pi
  Cy : Constant  Value=-0.018
  Gain : Gain  Gain=2
  Loa : Constant  Value=1.5
  Math Function : Math  Operator=magnitude^2  SignedPower=on
  Product : Product
  Product{1,3..6} (5 alike) : Product  Inputs=3
  Product2 : Product
  Sum : Sum  Inputs=|+--
  Trigonometric Function : Trigonometry
  Trigonometric Function1 : Trigonometry  Operator=cos
  Trigonometric Function2 : Trigonometry
  Wind Density : Constant  Value=1.225
  half : Constant  Value=0.5
  TeU : Outport
  TeV : Outport  Port=2
  TeR : Outport  Port=3
  wires:
  Vw/1 -> Math Function/1
  Product/1 -> TeU/1
  Afw/1 -> Product/1
  Product2/1 -> TeV/1
  Alw/1 -> Product2/1
  Product1/1 -> TeR/1
  Alw1/1 -> Product1/1
  Loa/1 -> Product1/3
  Yaw/1 -> Sum/1
  Beta/1 -> Sum/2
  Cx1/1 -> Sum/3
  Wind Density/1 -> Product3/2
  Math Function/1 -> Product3/3
  half/1 -> Product3/1
  Product4/1 -> Product/2
  Trigonometric Function1/1 -> Product4/2
  Cx/1 -> Product4/3
  Sum/1 -> Trigonometric Function1/1, Gain/1, Trigonometric Function/1
  Product3/1 -> Product6/1, Product5/1, Product4/1
  Product5/1 -> Product2/2
  Trigonometric Function/1 -> Product5/2
  Cy/1 -> Product5/3
  Product6/1 -> Product1/2
  Trigonometric Function2/1 -> Product6/2
  Cn/1 -> Product6/3
  Gain/1 -> Trigonometric Function2/1

== matlab function x3DOF_bener/Subsystem/ILOS Guidance ==
  settings: updateMethod=DISCRETE
  data: x input; psi_d output; x_e output; y input; Delta input; R_switch input; xdata input; ydata input; U input; K_f input; h input; y_e output; Gpi input; xk_next output; yk_next output; xk_ahead output; yk_ahead output; stop output
function [psi_d,x_e, y_e,xk_next,yk_next,xk_ahead,yk_ahead,stop]= fcn(x,y,Delta,R_switch,xdata,ydata,U,K_f,h,Gpi)

% waypoints
wpt.pos.x = xdata;
wpt.pos.y = ydata;

% ILOS guidance law
[psi_d,x_e,y_e,xk_next,yk_next,xk_ahead,yk_ahead,stop] = ILOSpsi(x,y,Delta,h,R_switch,wpt,U,K_f,Gpi);

end

== matlab function x3DOF_bener/Subsystem/LOS Guidance ==
  settings: updateMethod=DISCRETE
  data: x input; psi_d output; y input; Delta input; R_switch input; xdata input; ydata input; U input; K_f input; h input; x_e output; y_e output; flag output; Gpi input
function [psi_d,x_e, y_e,flag]= fcn(x,y,Delta,R_switch,xdata,ydata,U,K_f,h,Gpi)

% waypoints
wpt.pos.x = xdata;
wpt.pos.y = ydata;

% LOS guidance law
[psi_d,x_e,y_e,flag] = LOSpsi(x,y,Delta,h,R_switch,wpt,U,K_f,Gpi);

end

== matlab function x3DOF_bener/MATLAB Function1 ==
  data: Vx input; y output; Vy input
function y = fcn(Vx,Vy)

y = sqrt(Vx.^2+Vy.^2);

== matlab function x3DOF_bener/Fuzzy PID Yaw/MATLAB Function ==
  settings: updateMethod=DISCRETE  sampleTime=0.005
  data: Delta_Kp input; Kp output; Delta_Ki input; Delta_Kd input; Ki output; Kd output
function [Kp,Ki,Kd] = Delta_Gain_yaw(Delta_Kp,Delta_Ki,Delta_Kd)
    
    Kp_init = 8; Ki_init = 0; Kd_init = 6.5;
    
    Kp = Kp_init + Delta_Kp;
    Ki = Ki_init + Delta_Ki;
    Kd = Kd_init + Delta_Kd;
    if Kp < 0
        Kp = 0;
    end
    if Ki < 0
        Ki = 0;
    end
    if Kd < 0
        Kd = 0;
    end
end

== matlab function x3DOF_bener/Fuzzy PID Yaw/MATLAB Function1 ==
  data: Reference input; Error output; Error_In input
function Error = Checking_Mapping(Reference,Error_In)
    if Reference < 0
        Error = -1*Error_In;
    else
        Error = Error_In;
    end
    Error = wrapToPi(Error);

== matlab function x3DOF_bener/Fuzzy PID Yaw/MATLAB Function2 ==
  data: u input; y output
function y = fcn(u)

y = wrapToPi(u);

== matlab function x3DOF_bener/FLC Yaw/MATLAB Function1 ==
  data: Reference input; Error output; Error_In input
function Error = Checking_Mapping(Reference,Error_In)
    if Reference < 0
        Error = -1*Error_In;
    else
        Error = Error_In;
    end
    Error = wrapToPi(Error);

== matlab function x3DOF_bener/BACK UP TIDAK DIGUNAKAN/MATLAB Function2 ==
  settings: updateMethod=DISCRETE
  data: v_actual input; x_current input; x_next input; v_ref output; d_lookahead output; d_next output; v_normal input; t_lookahead input; psi_error output; psi_error input; turning_factor output; cte input
function [v_ref, d_lookahead, d_next, psi_error,turning_factor] = MATLAB_Function4(v_actual, x_current, x_next, v_normal, t_lookahead, psi_error,cte)
    % Parameter
    v_min = 0.05 * v_normal; % Kecepatan minimum
    v_stop = 0; % Kecepatan nol untuk koreksi yaw
    stop_threshold = deg2rad(10); % Threshold yaw error untuk berhenti
    stop_duration = 10; % Durasi berhenti (dalam langkah simulasi)
    d_next = norm(x_next - x_current); % Jarak ke waypoint berikutnya
    psi_error = abs(psi_error); % Error yaw dalam radian

    % Persistent timer untuk durasi saat v_ref = 0
    persistent stop_timer;
    if isempty(stop_timer)
        stop_timer = 0; % Inisialisasi timer
    end
    
    % Prediksi jarak lookahead
    d_lookahead = max(0.5, v_actual * t_lookahead); % Prediksi jarak tempuh minimum

    % Default nilai v_ref
    v_ref = v_normal; % Set nilai awal ke kecepatan normal
    turning_factor = 1;
    % Koreksi yaw besar: Hentikan sementara untuk mengoreksi
    if psi_error > stop_threshold
        v_ref = v_stop; % Kapal berhenti
        stop_timer = stop_timer + 1; % Hitung durasi
    else
        stop_timer = 0; % Reset timer jika yaw error kecil
    end

    % Setelah berhenti untuk durasi tertentu, kembali ke v_min
    if stop_timer > stop_duration
        v_ref = v_min; % Kembali ke kecepatan minimum
        stop_timer = 0; % Reset timer
    end

    % Jika yaw error kecil, gunakan turning_factor berbasis cos
    if psi_error <= stop_threshold
        turning_factor = max(cos(psi_error), 0.1); % Smooth transition
        if psi_error < deg2rad(5) % Jalur lurus
            turning_factor = 1;
        end

        % Perhitungkan jarak lookahead terhadap waypoint
        if d_lookahead > d_next && cte > abs(0.1)
            turning_factor = turning_factor * 0.5; % Kurangi kecepatan lebih lanjut
        end

        % Hitung v_ref dengan turning_factor
        v_ref = v_normal * turning_factor;
    end

    % Pastikan v_ref dalam batas
    v_ref = max(v_min, min(v_normal, v_ref));
end

== matlab function x3DOF_bener/Fuzzy PID Yaw1/MATLAB Function ==
  settings: updateMethod=DISCRETE  sampleTime=0.005
  data: Delta_Kp input; Kp output; Delta_Ki input; Delta_Kd input; Ki output; Kd output
function [Kp,Ki,Kd] = Delta_Gain_yaw(Delta_Kp,Delta_Ki,Delta_Kd)
    
    Kp_init = 4; Ki_init = 0; Kd_init = 6.5;
    
    Kp = Kp_init + Delta_Kp;
    Ki = Ki_init + Delta_Ki;
    Kd = Kd_init + Delta_Kd;
    if Kp < 0
        Kp = 0;
    end
    if Ki < 0
        Ki = 0;
    end
    if Kd < 0
        Kd = 0;
    end
end

== matlab function x3DOF_bener/Fuzzy PID Surge1/MATLAB Function ==
  settings: updateMethod=DISCRETE  sampleTime=0.005
  data: Delta_Kp input; Kp output; Delta_Ki input; Delta_Kd input; Ki output; Kd output
function [Kp,Ki,Kd] = Delta_Gain_surge(Delta_Kp,Delta_Ki,Delta_Kd)
    
    Kp_init = 25; Ki_init = 15; Kd_init = 1;
    
    Kp = Kp_init + Delta_Kp;
    Ki = Ki_init + Delta_Ki;
    Kd = Kd_init + Delta_Kd;
    if Kp < 0
        Kp = 0;
    end
    if Ki < 0
        Ki = 0;
    end
    if Kd < 0
        Kd = 0;
    end
end
